simulink model "sf_enabled_subsystem_temp_logic"  (R2025b)
settings: Solver=FixedStepDiscrete  StartTime=0.0  StopTime=12  FixedStep=0.01  RelTol=1e-3
libraries: SignalEditorBlockLib x1
settings Model: Creator=The MathWorks, Inc.  LastModifiedBy=The MathWorks, Inc.
settings SolverCC: AlgebraicLoopSolver=TrustRegion
settings DataIOCC: LimitDataPoints=on  SaveFormat=Array  ReturnWorkspaceOutputs=off
settings OptimizationCC: ReuseModelBlockBuffer=off  ExpressionDepthLimit=2147483647.0  InitFltsAndDblsToZero=on  LifeSpan=inf
settings DebuggingCC: UnderspecifiedInitializationDetection=Classic  MergeDetectMultiDrivingBlocksExec=none  SolverPrmCheckMsg=warning  FcnCallInpInsideContextMsg=warning  UnconnectedInputMsg=warning  UnconnectedOutputMsg=warning  UnconnectedLineMsg=warning  StateNameClashWarn=warning  SFUnexpectedBacktrackingDiag=warning  SFNoUnconditionalDefaultTransitionDiag=warning  SFExecutionAtInitializationDiag=none  ArithmeticOperatorsInVariantConditions=warning
settings HardwareCC: ProdBitPerPointer=32.0  ProdBitPerSizeT=32.0  ProdBitPerPtrDiffT=32.0  ProdLargestAtomicFloat=None  ProdIntDivRoundTo=Undefined  ProdEndianess=Unspecified  ProdWordSize=32.0  ProdHWDeviceType=32-bit Generic
settings ModelReferenceCC: EnableRefExpFcnMdlSchedulingChecks=on  PropagateSignalLabelsOutOfModel=off
settings SFSimCC: SimUseLocalCustomCode=off  SimParseCustomCode=off  CustomCodeUndefinedFunction=UseInterfaceOnly
settings RTWCC: RTWUseLocalCustomCode=off  GPUComputeCapability=3.5
settings CodeAppCC: StateflowObjectComments=on
settings GRTTargetCC: TargetLangStandard=C89/C90 (ANSI)  CombineOutputUpdateFcns=off  GRTInterface=on
settings ConfigComp: CovMetricSettings=dw  CovSaveCumulativeToWorkspaceVar=on  CovSaveSingleToWorkspaceVar=on  CovExternalEMLEnable=off

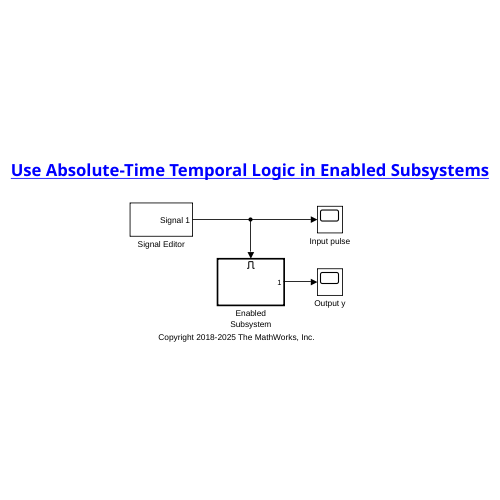
[thumbnail: Simulink's stored preview of the top-level diagram]
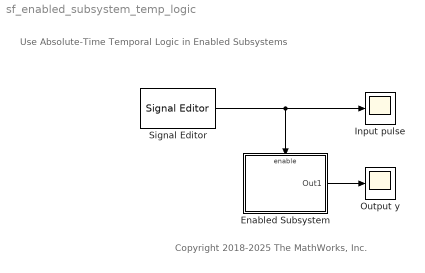
== system sf_enabled_subsystem_temp_logic ==
  note: Copyright 2018-2025 The MathWorks, Inc.
  note: Use Absolute-Time Temporal Logic in Enabled Subsystems
  Enabled Subsystem : Subsystem  TreatAsAtomicUnit=on
  Input pulse : Scope
      settings: ActiveDisplayYMinimum=-0.5  ActiveDisplayYMaximum=1.5
  Output y : Scope
      settings: ActiveDisplayYMinimum=-0.5  ActiveDisplayYMaximum=1.5
  Signal Editor : SignalEditorBlockLib/Signal Editor  FileName=enabled_subsystem_temp_logic.mat  ActiveScenario=Input_pulse  ActiveSignal=Signal 1  IsBus=off  OutputBusObjectStr=Bus: BusObject  SampleTime=0  OutputAfterFinalValue=Extrapolation  Unit=inherit  PreserveSignalName=on  ApplySigPropsToAllScenarios=on  ApplySigPropsToAllSignals=off  SignalPropertySource=Dialog parameters
  wires:
  Enabled Subsystem/1(Out1) -> Output y/1
  Signal Editor/1 -> Enabled Subsystem/Enable, Input pulse/1

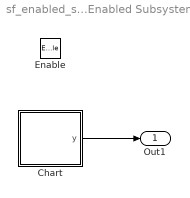
== system sf_enabled_subsystem_temp_logic/Enabled Subsystem ==
  Enable : EnablePort
  Chart : Stateflow chart  TreatAsAtomicUnit=on
  Out1 : Outport  VectorParamsAs1DForOutWhenUnconnected=off
  wires:
  Chart/1(y) -> Out1/1

== stateflow chart sf_enabled_subsystem_temp_logic/Enabled Subsystem/Chart ==
  settings: updateMethod=DISCRETE  sampleTime=0.01
  state A
    y = 0;
  state B
    y = 1;
  (default) -> A
  A -> B : after(5, sec)
  data: y output double
